simulink model "springdamper_model"  (R2020a)
settings: Solver=ode45  StartTime=0.0  StopTime=4  MaxStep=0.0009  MinStep=0.0001  RelTol=1e-3
values from neighbouring files (symbols this model uses):
  C_W = 1000    [springdamper_data.m]
  H_PC = 0.1265    [springdamper_data.m]
  H_RC_FRONT = 0.0346    [springdamper_data.m]
  H_RC_REAR = 0.0779    [springdamper_data.m]
  K_S = 26300    [springdamper_data.m]
  K_W = 50000    [springdamper_data.m]
  PC_TO_FRONT_AXLE = 0.667    [springdamper_data.m]
  PC_TO_REAR_AXLE = WHEELBASE-0.667    (= 0.873)    [springdamper_data.m]
  PITCH_INERTIA_PC = PITCH_INERTIA + SUSP_MASS*PC_TO_SUSPCOG^2    (= 73.7412)    [springdamper_data.m]
  pull = pull15431543    [springdamper_data.m]
  push = push15431543    [springdamper_data.m]
  QUARTER_MASS = 13    [springdamper_data.m]
  RC_TO_WHEEL_FRONT = TRACK_FRONT/2    (= 0.6)    [springdamper_data.m]
  RC_TO_WHEEL_REAR = TRACK_REAR/2    (= 0.58)    [springdamper_data.m]
  ROLL_INERTIA_RC = ROLL_INERTIA + SUSP_MASS*((RC_TO_SUSPCOG_FRONT+RC_TO_SUSPCOG_REAR)/2)^2    (= 22.694437)    [springdamper_data.m]
  SUSP_MASS = 208    [springdamper_data.m]
  SUSPCOG = 0.283    [springdamper_data.m]
  vel = [0 12.5 25 50 75 100 125 150 175 200 225 250]    [springdamper_data.m]
  WHEELBASE = 1.54    [springdamper_data.m]
  YAW_INERTIA = 63    [springdamper_data.m]
undefined symbols (not defined in the file or in its folder): sigbuilder_block
libraries: simulink_extras x6, simulink x3
(part 2 of 2)

== system springdamper_model/Roll_stiffness_from_springs2/rear_left ==
  Motion_ratio : Inport
  Divide1 : Product  Inputs=*/
  Spring_stiffness1 : Constant  Value=K_S
  Square1 : Math  Operator=square  SaturateOnIntegerOverflow=on
  rear_wheel_rate : Outport
  wires:
  Motion_ratio/1 -> Square1/1
  Spring_stiffness1/1 -> Divide1/1
  Square1/1 -> Divide1/2
  Divide1/1 -> rear_wheel_rate/1

== system springdamper_model/Roll_stiffness_from_springs2/rear_right ==
  Motion_ratio : Inport
  Divide1 : Product  Inputs=*/
  Spring_stiffness1 : Constant  Value=K_S
  Square1 : Math  Operator=square  SaturateOnIntegerOverflow=on
  rear_wheel_rate : Outport
  wires:
  Divide1/1 -> rear_wheel_rate/1
  Square1/1 -> Divide1/2
  Spring_stiffness1/1 -> Divide1/1
  Motion_ratio/1 -> Square1/1

== system springdamper_model/springs/front_left ==
  Motion_ratio : Inport
  Divide : Product  Inputs=*/
  Spring_stiffness : Constant  Value=K_S
  Square : Math  Operator=square  SaturateOnIntegerOverflow=on
  front_wheel_rate [N/m] : Outport
  wires:
  Square/1 -> Divide/2
  Motion_ratio/1 -> Square/1
  Spring_stiffness/1 -> Divide/1
  Divide/1 -> front_wheel_rate [N/m]/1

== system springdamper_model/springs/rear_left ==
  Motion_ratio : Inport
  Divide1 : Product  Inputs=*/
  Spring_stiffness1 : Constant  Value=K_S
  Square1 : Math  Operator=square  SaturateOnIntegerOverflow=on
  rear_wheel_rate : Outport
  wires:
  Square1/1 -> Divide1/2
  Motion_ratio/1 -> Square1/1
  Spring_stiffness1/1 -> Divide1/1
  Divide1/1 -> rear_wheel_rate/1

== system springdamper_model/springs1/front_left ==
  Motion_ratio : Inport
  Divide : Product  Inputs=*/
  Spring_stiffness : Constant  Value=K_S
  Square : Math  Operator=square  SaturateOnIntegerOverflow=on
  front_wheel_rate [N/m] : Outport
  wires:
  Square/1 -> Divide/2
  Motion_ratio/1 -> Square/1
  Spring_stiffness/1 -> Divide/1
  Divide/1 -> front_wheel_rate [N/m]/1

== system springdamper_model/springs1/rear_left ==
  Motion_ratio : Inport
  Divide1 : Product  Inputs=*/
  Spring_stiffness1 : Constant  Value=K_S
  Square1 : Math  Operator=square  SaturateOnIntegerOverflow=on
  rear_wheel_rate : Outport
  wires:
  Square1/1 -> Divide1/2
  Motion_ratio/1 -> Square1/1
  Spring_stiffness1/1 -> Divide1/1
  Divide1/1 -> rear_wheel_rate/1
